simulink model "Catmull_Rom_2025"  (R2023b)
settings: Solver=VariableStepDiscrete  StartTime=0.0  StopTime=20  MaxStep=0.02  RelTol=1e-3
values from neighbouring files (symbols this model uses):
  sim_IC_x = Spline_Ref_Poses(1,1)    [Catmull_Rom_2025_data.m]
  sim_IC_y = Spline_Ref_Poses(1,2)    [Catmull_Rom_2025_data.m]
  Spline_Num_Poses = All_Paths_Num_Poses(k)    [Catmull_Rom_2025_data.m]
  Spline_Ref_Poses = All_Paths_Ref_Poses(:,:,k)    [Catmull_Rom_2025_data.m]
undefined symbols (not defined in the file or in its folder): DiscIntNeverNeededParam, Spline_Capture_Radius, Spline_Lookahead_Dist, Spline_Velocity_Axis
libraries: simulink_extras x1
settings Model: Creator=ander  LastModifiedBy=ander

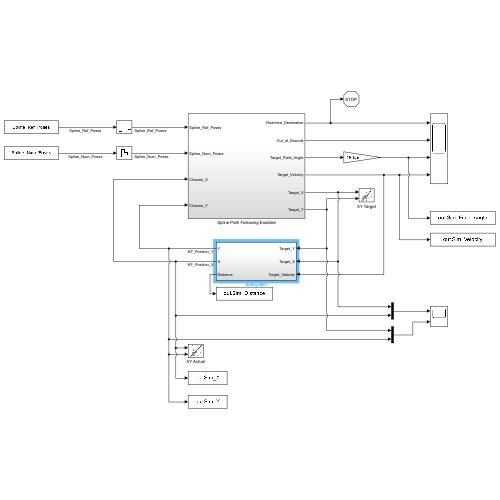
[thumbnail: Simulink's stored preview of the top-level diagram]
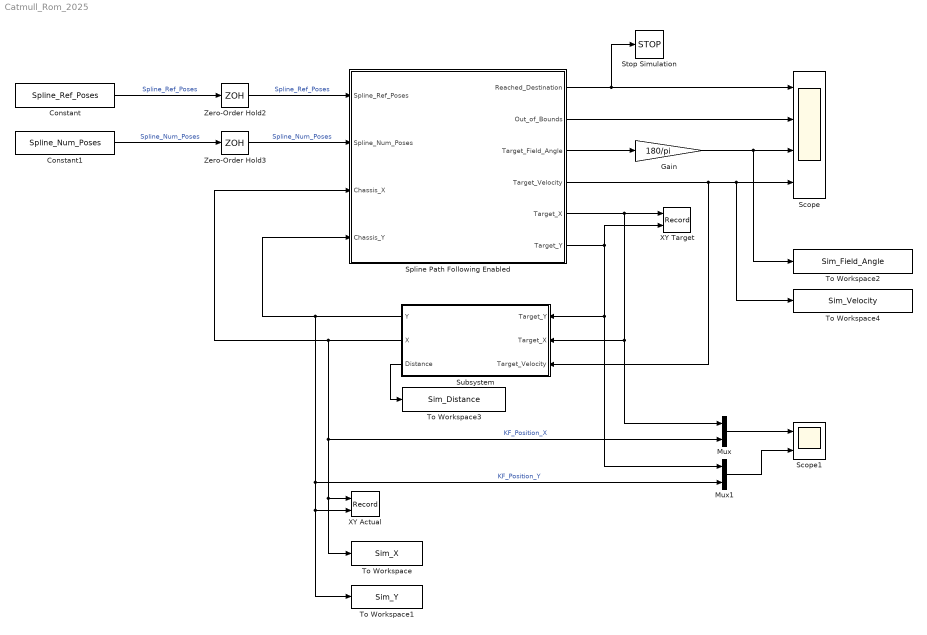
== system Catmull_Rom_2025 ==
  Constant : Constant  Value=Spline_Ref_Poses
  Constant1 : Constant  Value=Spline_Num_Poses
  Gain : Gain  Gain=180/pi
  Mux : Mux  Inputs=2
  Mux1 : Mux  Inputs=2
  Scope : Scope  NumInputPorts=4
  Scope1 : Scope  NumInputPorts=2
  Spline Path Following Enabled : Subsystem
  Stop Simulation : Stop
  Subsystem : Subsystem
  To Workspace : ToWorkspace  VariableName=Sim_X  SaveFormat=Structure With Time  SampleTime=0.02
      settings: Save2DSignal=2-D array (concatenate along first dimension)
  To Workspace1 : ToWorkspace  VariableName=Sim_Y  SaveFormat=Structure With Time  SampleTime=0.02
      settings: Save2DSignal=2-D array (concatenate along first dimension)
  To Workspace2 : ToWorkspace  VariableName=Sim_Field_Angle  SaveFormat=Structure With Time  SampleTime=0.02
      settings: Save2DSignal=2-D array (concatenate along first dimension)
  To Workspace3 : ToWorkspace  VariableName=Sim_Distance  SaveFormat=Structure With Time  SampleTime=0.02
      settings: Save2DSignal=2-D array (concatenate along first dimension)
  To Workspace4 : ToWorkspace  VariableName=Sim_Velocity  SaveFormat=Structure With Time  SampleTime=0.02
      settings: Save2DSignal=2-D array (concatenate along first dimension)
  XY Actual : Record  FileSettingsInternal="{\"entries\":[{\"content\":{\"excelSettings\":{\"content\":{},\"type\":\"Streamout.ExcelSettings\"}},\"type\":\"Streamout.FileSettingStorage\",\"uuid\":\"\"}],\"packageUris\":[\"http:\\/\\/schema.mathworks.com\\/mf0\\/streamout_blocks\\/R2020a\"],\"version\":\"1.0\"}"  Layout=[1 1]  SignalsInternal="{\"entries\":[{\"content\":{\"signals\":[{\"content\":{\"blockPath\":[],\"dimensions\":[1],\"domain\":\"\",\"lineColor\":\"#0072bd\",\"plots\":[1],\"port\":1,\"sid\":[\"\"],\"signalID\":10166,\"signalName\":\"KF_Position_X\"},\"type\":\"RecordBlkView.Signal\",\"uuid\":\"\"},{\"content\":{\"blockPath\":[],\"dimensions\":[1],\"domain\":\"\",\"lineColor\":\"#d95319\",\"plots\":[1],\"port\":2,\"sid\":[\"\"],\"signalID\":10170,\"signalName\":\"KF_Position_Y\"},\"type\":\"RecordBlkView.Signal\",\"uuid\":\"\"}]},\"type\":\"RecordBlkView.InputSignals\",\"uuid\":\"\"}],\"packageUris\":[\"http:\\/\\/schema.mathworks.com\\/mf0\\/streamout_blocks\\/R2020a\"],\"version\":\"1.0\"}"  VisualizationBindings="{\"xyplotplugin\":{\"info\":[{\"series\":[{\"bindingParametersList\":[{\"parameter\":\"X-Axis\",\"signalID\":10166,\"signalName\":\"KF_Position_X\"},{\"parameter\":\"Y-Axis\",\"signalID\":10170,\"signalName\":\"KF_Position_Y\"}],\"seriesID\":21168}],\"subplotID\":1}]}}"  CompatibilityTag=XY
  XY Target : Record  FileSettingsInternal="{\"entries\":[{\"content\":{\"excelSettings\":{\"content\":{},\"type\":\"Streamout.ExcelSettings\"}},\"type\":\"Streamout.FileSettingStorage\",\"uuid\":\"\"}],\"packageUris\":[\"http:\\/\\/schema.mathworks.com\\/mf0\\/streamout_blocks\\/R2020a\"],\"version\":\"1.0\"}"  Layout=[1 1]  SignalsInternal="{\"entries\":[{\"content\":{\"signals\":[{\"content\":{\"blockPath\":[],\"dimensions\":[1,1],\"domain\":\"\",\"lineColor\":\"#edb120\",\"plots\":[1],\"port\":1,\"sid\":[\"\"],\"signalID\":10174,\"signalName\":\"Spline Path Following Enabled:5\"},\"type\":\"RecordBlkView.Signal\",\"uuid\":\"\"},{\"content\":{\"blockPath\":[],\"dimensions\":[1,1],\"domain\":\"\",\"lineColor\":\"#7e2f8e\",\"plots\":[1],\"port\":2,\"sid\":[\"\"],\"signalID\":10178,\"signalName\":\"Spline Path Following Enabled:6\"},\"type\":\"RecordBlkView.Signal\",\"uuid\":\"\"}]},\"type\":\"RecordBlkView.InputSignals\",\"uuid\":\"\"}],\"packageUris\":[\"http:\\/\\/schema.mathworks.com\\/mf0\\/streamout_blocks\\/R2020a\"],\"version\":\"1.0\"}"  VisualizationBindings="{\"xyplotplugin\":{\"info\":[{\"series\":[{\"bindingParametersList\":[{\"parameter\":\"X-Axis\",\"signalID\":10174,\"signalName\":\"Spline Path Following Enabled:5\"},{\"parameter\":\"Y-Axis\",\"signalID\":10178,\"signalName\":\"Spline Path Following Enabled:6\"}],\"seriesID\":49111}],\"subplotID\":1}]}}"  CompatibilityTag=XY
  Zero-Order Hold2 : ZeroOrderHold  SampleTime=0.02
  Zero-Order Hold3 : ZeroOrderHold  SampleTime=0.02
  wires:
  Spline Path Following Enabled/1(Reached_Destination) -> Stop Simulation/1, Scope/1
  Spline Path Following Enabled/2(Out_of_Bounds) -> Scope/2
  Spline Path Following Enabled/3(Target_Field_Angle) -> Gain/1
  Spline Path Following Enabled/4(Target_Velocity) -> Subsystem/3(Target_Velocity), To Workspace4/1, Scope/4
  Constant/1 -> Zero-Order Hold2/1  "Spline_Ref_Poses"
  Constant1/1 -> Zero-Order Hold3/1  "Spline_Num_Poses"
  Zero-Order Hold2/1 -> Spline Path Following Enabled/1(Spline_Ref_Poses)  "Spline_Ref_Poses"
  Zero-Order Hold3/1 -> Spline Path Following Enabled/2(Spline_Num_Poses)  "Spline_Num_Poses"
  Subsystem/1(Y) -> Mux1/2, To Workspace1/1, XY Actual/2, Spline Path Following Enabled/4(Chassis_Y)  "KF_Position_Y"
  Subsystem/2(X) -> Mux/2, To Workspace/1, XY Actual/1, Spline Path Following Enabled/3(Chassis_X)  "KF_Position_X"
  Spline Path Following Enabled/6(Target_Y) -> Mux1/1, Subsystem/1(Target_Y), XY Target/2
  Spline Path Following Enabled/5(Target_X) -> Mux/1, Subsystem/2(Target_X), XY Target/1
  Mux/1 -> Scope1/1
  Mux1/1 -> Scope1/2
  Gain/1 -> To Workspace2/1, Scope/3
  Subsystem/3(Distance) -> To Workspace3/1

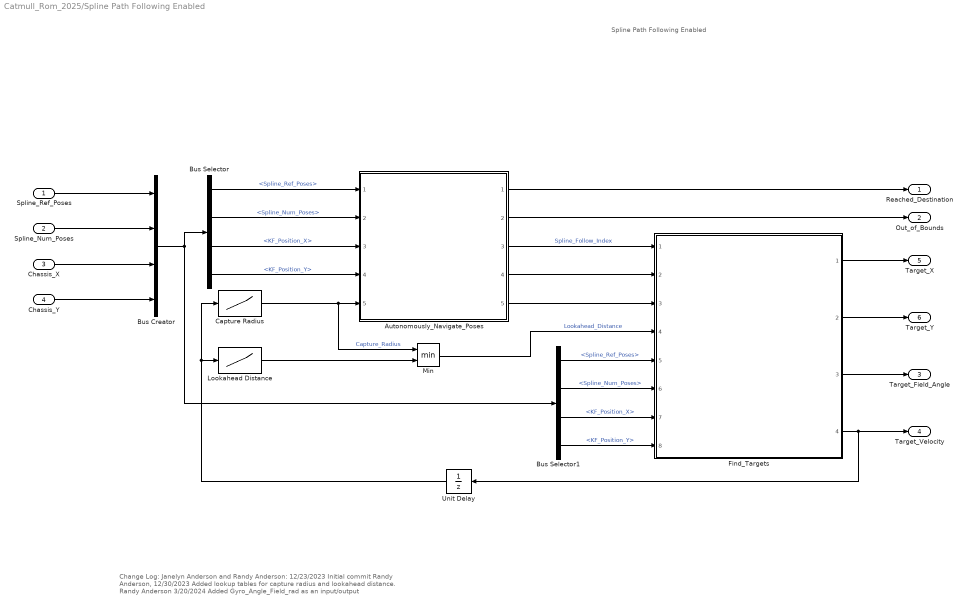
== system Catmull_Rom_2025/Spline Path Following Enabled ==
  note: Spline Path Following Enabled
  note: Change Log:
      | Janelyn Anderson and Randy Anderson: 12/23/2023
      | Initial commit
      | Randy Anderson, 12/30/2023
      | Added lookup tables for capture radius and lookahead distance.
      | Randy Anderson 3/20/2024
      | Added Gyro_Angle_Field_rad as an input/output
  Spline_Ref_Poses : Inport
  Spline_Num_Poses : Inport  Port=2
  Chassis_X : Inport  Port=3
  Chassis_Y : Inport  Port=4
  Autonomously_Navigate_Poses : Subsystem  ReferencedSubsystem=Autonomously_Navigate_Poses
  Bus Creator : BusCreator  Inputs=4
  Bus Selector : BusSelector  OutputSignals=Spline_Ref_Poses,Spline_Num_Poses,KF_Position_X,KF_Position_Y
  Bus Selector1 : BusSelector  OutputSignals=Spline_Ref_Poses,Spline_Num_Poses,KF_Position_X,KF_Position_Y
  Capture Radius : Lookup_n-D  NumberOfTableDimensions=1  BreakpointsForDimension1=Spline_Velocity_Axis  Table=Spline_Capture_Radius  ExtrapMethod=Clip  InternalRulePriority=Speed  RndMeth=Simplest
  Find_Targets : Subsystem  ReferencedSubsystem=Find_Target_Position_Velocity_Heading
  Lookahead Distance : Lookup_n-D  NumberOfTableDimensions=1  BreakpointsForDimension1=Spline_Velocity_Axis  Table=Spline_Lookahead_Dist  ExtrapMethod=Clip  InternalRulePriority=Speed  RndMeth=Simplest
  Min : MinMax  Inputs=2
  Unit Delay : UnitDelay  SampleTime=-1  HasFrameUpgradeWarning=on
  Reached_Destination : Outport
  Out_of_Bounds : Outport  Port=2
  Target_Field_Angle : Outport  Port=3
  Target_Velocity : Outport  Port=4
  Target_X : Outport  Port=5
  Target_Y : Outport  Port=6
  wires:
  Autonomously_Navigate_Poses/5 -> Find_Targets/3
  Autonomously_Navigate_Poses/4 -> Find_Targets/2
  Autonomously_Navigate_Poses/3 -> Find_Targets/1  "Spline_Follow_Index"
  Find_Targets/4 -> Target_Velocity/1, Unit Delay/1
  Spline_Ref_Poses/1 -> Bus Creator/1
  Spline_Num_Poses/1 -> Bus Creator/2
  Chassis_X/1 -> Bus Creator/3
  Chassis_Y/1 -> Bus Creator/4
  Bus Creator/1 -> Bus Selector1/1, Bus Selector/1
  Bus Selector/2 -> Autonomously_Navigate_Poses/2  "<Spline_Num_Poses>"
  Bus Selector/1 -> Autonomously_Navigate_Poses/1  "<Spline_Ref_Poses>"
  Bus Selector1/2 -> Find_Targets/6  "<Spline_Num_Poses>"
  Bus Selector1/1 -> Find_Targets/5  "<Spline_Ref_Poses>"
  Bus Selector/3 -> Autonomously_Navigate_Poses/3  "<KF_Position_X>"
  Bus Selector/4 -> Autonomously_Navigate_Poses/4  "<KF_Position_Y>"
  Bus Selector1/3 -> Find_Targets/7  "<KF_Position_X>"
  Bus Selector1/4 -> Find_Targets/8  "<KF_Position_Y>"
  Capture Radius/1 -> Autonomously_Navigate_Poses/5, Min/1  "Capture_Radius"
  Unit Delay/1 -> Lookahead Distance/1, Capture Radius/1
  Lookahead Distance/1 -> Min/2
  Min/1 -> Find_Targets/4  "Lookahead_Distance"
  Find_Targets/1 -> Target_X/1
  Find_Targets/2 -> Target_Y/1
  Find_Targets/3 -> Target_Field_Angle/1
  Autonomously_Navigate_Poses/1 -> Reached_Destination/1
  Autonomously_Navigate_Poses/2 -> Out_of_Bounds/1

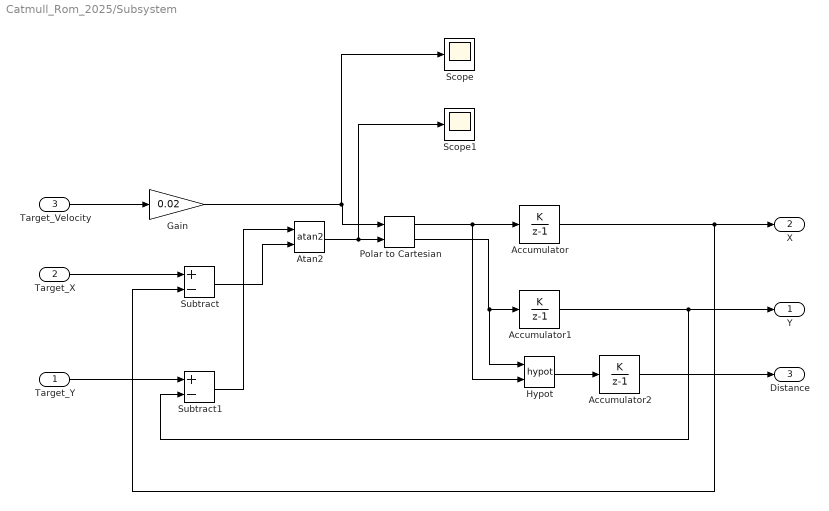
== system Catmull_Rom_2025/Subsystem ==
  Target_Y : Inport
  Target_X : Inport  Port=2
  Target_Velocity : Inport  Port=3
  Accumulator : DiscreteIntegrator  IntegratorMethod=Accumulation: Forward Euler  InitialCondition=sim_IC_x  SampleTime=-1  ICPrevOutput=DiscIntNeverNeededParam  ICPrevScaledInput=DiscIntNeverNeededParam
  Accumulator1 : DiscreteIntegrator  IntegratorMethod=Accumulation: Forward Euler  InitialCondition=sim_IC_y  SampleTime=-1  ICPrevOutput=DiscIntNeverNeededParam  ICPrevScaledInput=DiscIntNeverNeededParam
  Accumulator2 : DiscreteIntegrator  IntegratorMethod=Accumulation: Forward Euler  SampleTime=-1  ICPrevOutput=DiscIntNeverNeededParam  ICPrevScaledInput=DiscIntNeverNeededParam
  Atan2 : Trigonometry  Operator=atan2
  Gain : Gain  Gain=0.02
  Hypot : Math  Operator=hypot
  Polar to Cartesian : simulink_extras/Transformations/Polar to Cartesian
  Scope : Scope
  Scope1 : Scope
  Subtract : Sum  Inputs=+-
  Subtract1 : Sum  Inputs=+-
  Y : Outport
  X : Outport  Port=2
  Distance : Outport  Port=3
  wires:
  Target_X/1 -> Subtract/1
  Target_Y/1 -> Subtract1/1
  Subtract1/1 -> Atan2/1
  Subtract/1 -> Atan2/2
  Atan2/1 -> Scope1/1, Polar to Cartesian/2
  Target_Velocity/1 -> Gain/1
  Polar to Cartesian/1 -> Hypot/2, Accumulator/1
  Gain/1 -> Scope/1, Polar to Cartesian/1
  Polar to Cartesian/2 -> Hypot/1, Accumulator1/1
  Accumulator1/1 -> Y/1, Subtract1/2
  Accumulator/1 -> X/1, Subtract/2
  Hypot/1 -> Accumulator2/1
  Accumulator2/1 -> Distance/1
